simulink model "IDA_PBC"  (R2022b)
settings: Solver=FixedStepAuto  StartTime=0.0  StopTime=50  FixedStep=0.001  RelTol=1e-3
undefined symbols (not defined in the file): l_v, m_v, M_v, phi_desired, q2, q2_s
settings Model: Creator=ali14  LastModifiedBy=ali14

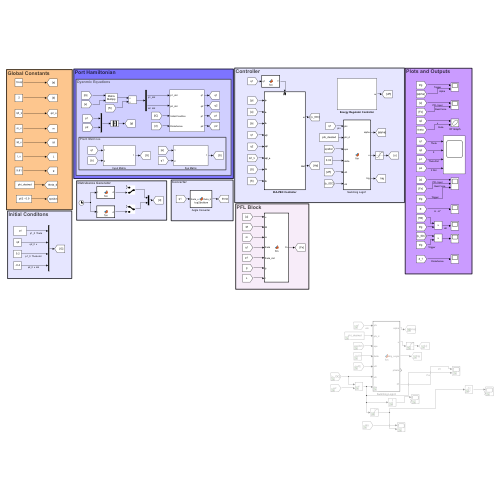
[thumbnail: Simulink's stored preview of the top-level diagram]
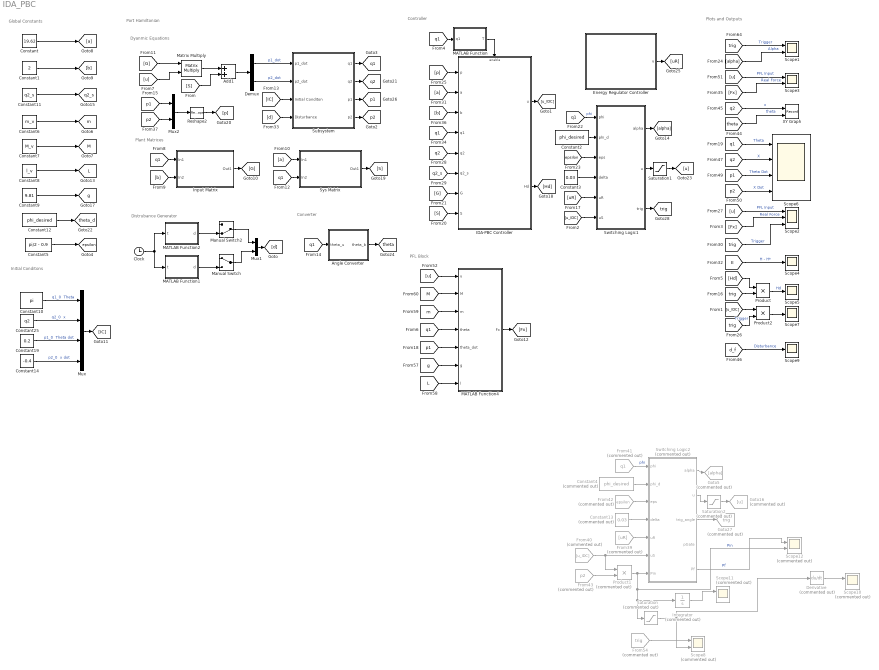
== system IDA_PBC ==
  note: Controller
  note: Plots and Outputs
  note: Initial Conditons
  note: Plant Matrices
  note: Dyanmic Equations
  note: Port Hamiltonian
  note: Converter
  note: Global Constants
  note: PFL Block
  note: Distrubance Generator
  Add1 : Sum
  Angle Converter : MATLAB Function  TreatAsAtomicUnit=on
  Clock : Clock
  Constant : Constant  Value=19.62
  Constant1 : Constant  Value=2
  Constant10 : Constant  Value=pi
  Constant11 : Constant  Value=q2_s
  Constant12 : Constant  Value=phi_desired
  Constant13 : Constant  Commented=on  Value=0.03
  Constant14 : Constant  Value=-0.4
  Constant19 : Constant  Value=0.2
  Constant2 : Constant  Value=phi_desired
  Constant25 : Constant  Value=q2
  Constant3 : Constant  Value=0.03
  Constant4 : Constant  Commented=on  Value=phi_desired
  Constant5 : Constant  Value=pi/2 - 0.9
  Constant6 : Constant  Value=m_v
  Constant7 : Constant  Value=M_v
  Constant8 : Constant  Value=l_v
  Constant9 : Constant  Value=9.81
  Demux : Demux  Outputs=2
  Derivative : Derivative  Commented=on
  Energy Regulator Controller : Subsystem
  From39 : From  Commented=on  GotoTag=uR
  From40 : From  Commented=on  GotoTag=u_IDC
  From41 : From  Commented=on  GotoTag=q1  TagVisibility=global
  From42 : From  Commented=on  GotoTag=epsilon  TagVisibility=global
  From43 : From  Commented=on  GotoTag=p2  TagVisibility=global
  From54 : From  Commented=on  GotoTag=trig  TagVisibility=global
  Goto16 : Goto  Commented=on  GotoTag=u
  Goto27 : Goto  Commented=on  GotoTag=trig  TagVisibility=global
  Goto5 : Goto  Commented=on  GotoTag=alpha
  IDA-PBC Controller : Subsystem
  Input Matrix : Subsystem
  Integrator : Integrator  Commented=on
  MATLAB Function : MATLAB Function  TreatAsAtomicUnit=on
  MATLAB Function1 : MATLAB Function  TreatAsAtomicUnit=on
  MATLAB Function2 : MATLAB Function  TreatAsAtomicUnit=on
  MATLAB Function4 : MATLAB Function  TreatAsAtomicUnit=on
  Manual Switch : ManualSwitch
  Manual Switch2 : ManualSwitch  CurrentSetting=0
  Matrix Multiply : Product  Multiplication=Matrix(*)
  Mux : Mux
  Mux1 : Mux  Inputs=2
  Mux2 : Mux  Inputs=2
  Product : Product
  Product1 : Product  Commented=on
  Product2 : Product
  Reshape2 : Reshape  OutputDimensionality=Column vector (2-D)
  Saturation : Saturate  Commented=on  UpperLimit=30  LowerLimit=-30
  Saturation1 : Saturate  UpperLimit=10  LowerLimit=-10
  Saturation2 : Saturate  Commented=on  UpperLimit=10  LowerLimit=-10
  Scope1 : Scope  NumInputPorts=2
  Scope{8,10..12} (4 alike) : Scope  Commented=on  NumInputPorts=2
  Scope2 : Scope  NumInputPorts=3
  Scope3 : Scope  NumInputPorts=2
  Scope{4..5,7,9} (4 alike) : Scope
  Scope6 : Scope  NumInputPorts=4
  Subsystem : Subsystem
  Switching Logic1 : MATLAB Function  TreatAsAtomicUnit=on
  Switching Logic2 : MATLAB Function  Commented=on  TreatAsAtomicUnit=on
  Sys Matrix : Subsystem
  XY Graph : Record  FileSettingsInternal="{\"entries\":[{\"content\":{\"excelSettings\":{\"content\":{},\"type\":\"Streamout.ExcelSettings\"}},\"type\":\"Streamout.FileSettingStorage\",\"uuid\":\"b4495491-268c-4705-8b0b-045f781b1a9d\"}],\"packageUris\":[\"http://schema.mathworks.com/mf0/streamout_blocks/R2020a\"],\"version\":\"1.0\"}"  Layout=[1 1]  SignalsInternal="{\"entries\":[{\"content\":{\"signals\":[{\"content\":{\"blockPath\":[\"IDA_PBC/XY Graph\"],\"channel\":[],\"dimensions\":[1,1],\"domain\":\"IDA_PBC/XY Graph\",\"lineColor\":\"#a2142f\",\"plots\":[1],\"port\":1,\"sid\":[\"\"],\"signalID\":19,\"signalName\":\"x\"},\"type\":\"RecordBlkView.Signal\",\"uuid\":\"3616e9f1-c643-483d-881a-894239690917\"},{\"content\":{\"blockPath\":[\"IDA_PBC/XY Graph\"],\"channel\":[],\"dimensions\":[1],\"domain\":\"IDA_PBC/XY Graph\",\"lineColor\":\"#139fff\",\"plots\":[1],\"port\":2,\"sid\":[\"\"],\"signalID\":23,\"signalName\":\"theta\"},\"type\":\"RecordBlkView.Signal\",\"uuid\":\"444c35d6-5370-4ebf-81a1-b594d5e0da69\"}]},\"type\":\"RecordBlkView.InputSignals\",\"uuid\":\"ab54f437-3e6c-482a-a295-04311a9801ac\"}],\"packageUris\":[\"http://schema.mathworks.com/mf0/streamout_blocks/R2020a\"],\"version\":\"1.0\"}"  VisualizationBindings="{\"xyplotplugin\":{\"info\":[{\"series\":[{\"bindingParametersList\":[{\"parameter\":\"X-Axis\",\"signalID\":19,\"signalName\":\"x\"},{\"parameter\":\"Y-Axis\",\"signalID\":23,\"signalName\":\"theta\"}],\"seriesID\":56537}],\"subplotID\":1}]}}"  CompatibilityTag=XY
  tag scope: L=global, M=global, epsilon=global, g=global, m=global, p1=global, p2=global, q1=global, q2=global, q2_s=global, theta=global, theta_d=global, trig=global
  wires:
  Constant/1 -> [a]
  Constant1/1 -> [b]
  [G] -> Matrix Multiply/1
  [u] -> Matrix Multiply/2
  Matrix Multiply/1 -> Add1/1
  Add1/1 -> Demux/1
  Constant11/1 -> [q2_s]
  [q2] -> XY Graph/1  "x"
  [theta] -> XY Graph/2  "theta"
  [q1] -> Scope6/1  "Theta"
  [q2] -> Scope6/2  "X"
  [p1] -> Scope6/3  "Theta Dot"
  [p2] -> Scope6/4  "X Dot"
  [u] -> Scope3/1  "PFL Input"
  [m] -> MATLAB Function4/3(m)
  [L] -> MATLAB Function4/7(l)
  [p1] -> MATLAB Function4/5(theta_dot)
  [g] -> MATLAB Function4/6(g)
  [q1] -> MATLAB Function4/4(theta)
  [M] -> MATLAB Function4/2(M)
  [u] -> MATLAB Function4/1(u)
  MATLAB Function4/1(Fx) -> [Fx]
  [G] -> IDA-PBC Controller/7(G)
  [S] -> IDA-PBC Controller/8(S)
  [p] -> IDA-PBC Controller/1(p)
  [a] -> IDA-PBC Controller/2(a)
  [b] -> IDA-PBC Controller/3(b)
  [q2_s] -> IDA-PBC Controller/6(q2_s)
  Constant7/1 -> [M]
  Constant6/1 -> [m]
  Constant8/1 -> [L]
  Constant9/1 -> [g]
  Constant12/1 -> [theta_d]
  [q1] -> Angle Converter/1(theta_u)
  Angle Converter/1(theta_b) -> [theta]
  Mux2/1 -> Reshape2/1
  Reshape2/1 -> [p]
  [p1] -> Mux2/1
  [p2] -> Mux2/2
  MATLAB Function/1(T) -> IDA-PBC Controller/Enable
  Constant5/1 -> [epsilon]
  IDA-PBC Controller/1(u) -> [u_IDC]
  [q1] -> Input Matrix/1(In1)
  [b] -> Input Matrix/2(In2)
  Input Matrix/1(Out1) -> [G]
  [a] -> Sys Matrix/1(In1)
  [q1] -> Sys Matrix/2(In2)
  Sys Matrix/1(Out1) -> [S]
  [S] -> Add1/2
  Constant25/1 -> Mux/2  "q2_0  x"
  Constant10/1 -> Mux/1  "q1_0  Theta"
  Constant19/1 -> Mux/3  "p1_0  Theta dot"
  Constant14/1 -> Mux/4  "p2_0  x dot"
  Subsystem/4(p2) -> [p2]
  Subsystem/2(q2) -> [q2]
  Subsystem/3(p1) -> [p1]
  Subsystem/1(q1) -> [q1]
  Mux/1 -> [IC]
  [IC] -> Subsystem/3(Initial Conditon)
  Demux/1 -> Subsystem/1(p1_dot)  "p1_dot"
  Demux/2 -> Subsystem/2(p2_dot)  "p2_dot"
  MATLAB Function2/1(d) -> Manual Switch2/2
  Manual Switch2/1 -> Mux1/1
  MATLAB Function1/1(d) -> Manual Switch/2
  Manual Switch/1 -> Mux1/2
  Clock/1 -> MATLAB Function2/1(t), MATLAB Function1/1(t)
  Mux1/1 -> [d]
  [d] -> Subsystem/4(Disturbance)
  [Fx] -> Scope3/2  "Real Force"
  [q1] -> IDA-PBC Controller/4(q1)
  [q2] -> IDA-PBC Controller/5(q2)
  Energy Regulator Controller/1(u) -> [uR]
  IDA-PBC Controller/2(Hd) -> [Hd]
  [q1] -> MATLAB Function/1(q1)
  Constant2/1 -> Switching Logic1/2(phi_d)
  Switching Logic1/2(u) -> Saturation1/1
  [epsilon] -> Switching Logic1/3(eps)
  Switching Logic1/1(alpha) -> [alpha]
  [q1] -> Switching Logic1/1(phi)  "phi"
  [uR] -> Switching Logic1/5(uR)
  [u_IDC] -> Switching Logic1/6(uS)
  Constant3/1 -> Switching Logic1/4(delta)
  [trig] -> Scope1/1  "Trigger"
  Switching Logic1/3(trig) -> [trig]
  [alpha] -> Scope1/2  "Alpha"
  [Fx] -> Scope2/2  "Real Force"
  [u] -> Scope2/1  "PFL Input"
  [trig] -> Scope2/3  "Trigger"
  [E] -> Scope4/1  "H - H*"
  Product/1 -> Scope5/1  "Hd"
  [trig] -> Product/2
  [Hd] -> Product/1
  Saturation1/1 -> [u]
  Switching Logic2/2(u) -> Saturation2/1
  Saturation2/1 -> Goto16/1
  From41/1 -> Switching Logic2/1(phi)  "phi"
  Constant13/1 -> Switching Logic2/4(delta)
  Switching Logic2/1(alpha) -> Goto5/1
  From39/1 -> Switching Logic2/5(uR)
  Switching Logic2/3(trig_angle) -> Goto27/1
  Constant4/1 -> Switching Logic2/2(phi_d)
  From40/1 -> Switching Logic2/6(uS), Product1/1
  From42/1 -> Switching Logic2/3(eps)
  Product1/1 -> Scope12/2, Integrator/1, Saturation/1, Switching Logic2/7(Pin)  "Pin"
  From43/1 -> Product1/2
  Saturation/1 -> Derivative/1, Scope8/2
  From54/1 -> Scope8/1
  Derivative/1 -> Scope10/1
  Integrator/1 -> Scope11/1
  Switching Logic2/5(Pf) -> Scope12/1  "Pf"
  [u_IDC] -> Product2/1
  [trig] -> Product2/2  "Trigger"
  Product2/1 -> Scope7/1
  [d_f] -> Scope9/1  "Disturbance"

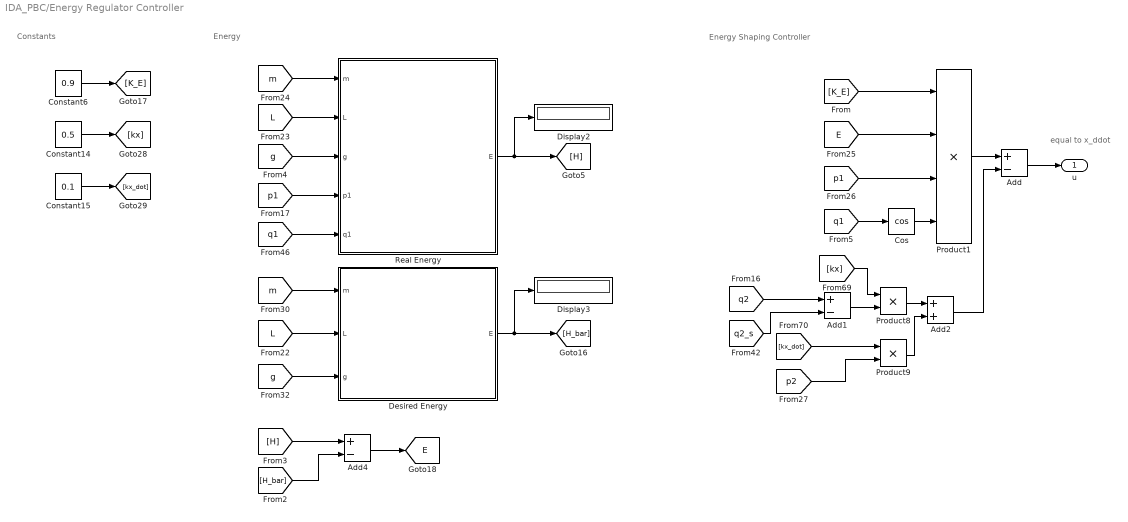
== system IDA_PBC/Energy Regulator Controller ==
  note: Energy
  note: Energy Shaping Controller
  note: Constants
  note: equal to x_ddot
  Add : Sum  Inputs=+-
  Add1 : Sum  Inputs=+-
  Add2 : Sum
  Add4 : Sum  Inputs=+-
  Constant14 : Constant  Value=0.5
  Constant15 : Constant  Value=0.1
  Constant6 : Constant  Value=0.9
  Cos : Trigonometry  Operator=cos
  Desired Energy : Subsystem
  Display2 : Display
  Display3 : Display
  Product1 : Product  Inputs=4
  Product8 : Product
  Product9 : Product
  Real Energy : Subsystem
  u : Outport
  tag scope: E=global
  wires:
  [H_bar] -> Add4/2
  [g] -> Real Energy/3(g)
  Real Energy/1(E) -> [H], Display2/1
  [m] -> Real Energy/1(m)
  [q1] -> Real Energy/5(q1)
  Desired Energy/1(E) -> [H_bar], Display3/1
  [L] -> Desired Energy/2(L)
  [m] -> Desired Energy/1(m)
  [L] -> Real Energy/2(L)
  [H] -> Add4/1
  Add4/1 -> [E]
  [p1] -> Real Energy/4(p1)
  [g] -> Desired Energy/3(g)
  Add/1 -> u/1
  [q2_s] -> Add1/2
  [q2] -> Add1/1
  Add1/1 -> Product8/2
  Constant15/1 -> [kx_dot]
  Constant14/1 -> [kx]
  Add2/1 -> Add/2
  [K_E] -> Product1/1
  [E] -> Product1/2
  [p1] -> Product1/3
  [kx_dot] -> Product9/1
  Product1/1 -> Add/1
  Constant6/1 -> [K_E]
  Cos/1 -> Product1/4
  [p2] -> Product9/2
  [kx] -> Product8/1
  Product9/1 -> Add2/2
  Product8/1 -> Add2/1
  [q1] -> Cos/1

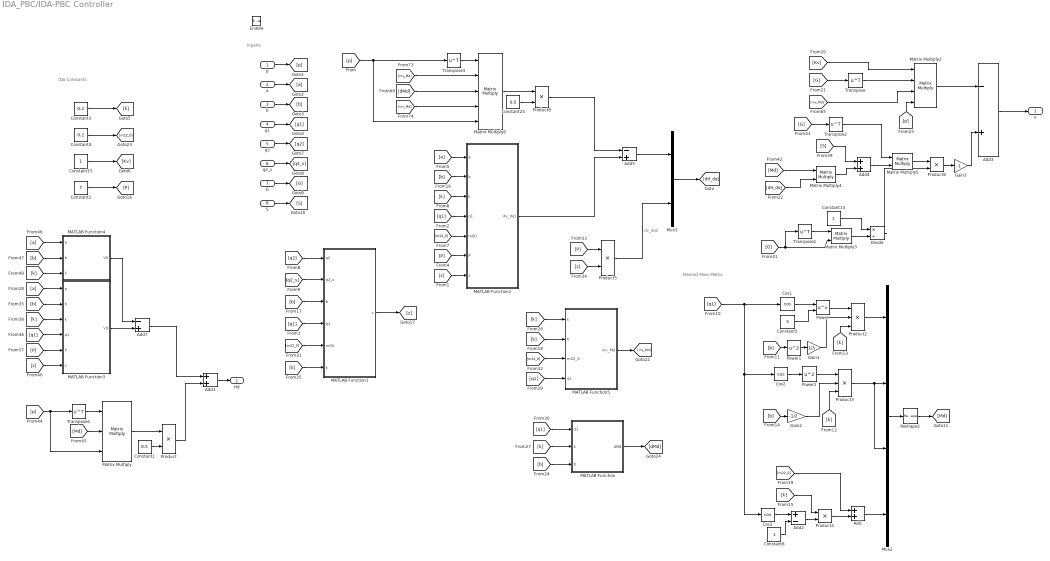
== system IDA_PBC/IDA-PBC Controller ==
  note: Inports
  note: Desired Mass Matrix
  note: IDA Constants
  p : Inport
  a : Inport  Port=2
  b : Inport  Port=3
  q1 : Inport  Port=4
  q2 : Inport  Port=5
  q2_s : Inport  Port=6
  G : Inport  Port=7
  S : Inport  Port=8
  Enable : EnablePort
  Add : Sum
  Add1 : Sum
  Add2 : Sum  Inputs=+-
  Add3 : Sum  Inputs=-+
  Add4 : Sum
  Add5 : Sum  Inputs=-+
  Add7 : Sum  Inputs=-+
  Constant1 : Constant  Value=0.5
  Constant13 : Constant
  Constant15 : Constant
  Constant2 : Constant  Value=7
  Constant24 : Constant  Value=0.5
  Constant3 : Constant  Value=0.2
  Constant4 : Constant  Value=0.2
  Constant5 : Constant  Value=3
  Constant8 : Constant
  Cos1 : Trigonometry  Operator=cos
  Cos2 : Trigonometry  Operator=cos
  Cos3 : Trigonometry  Operator=cos
  Divide : Product  Inputs=*/
  Gain1 : Gain  Gain=1/3
  Gain2 : Gain  Gain=-1/2
  Gain3 : Gain  Gain=-1
  MATLAB Function : MATLAB Function  TreatAsAtomicUnit=on
  MATLAB Function1 : MATLAB Function  TreatAsAtomicUnit=on
  MATLAB Function2 : MATLAB Function  TreatAsAtomicUnit=on
  MATLAB Function3 : MATLAB Function  TreatAsAtomicUnit=on
  MATLAB Function4 : MATLAB Function  TreatAsAtomicUnit=on
  MATLAB Function5 : MATLAB Function  TreatAsAtomicUnit=on
  Matrix Multiply : Product  Inputs=3  Multiplication=Matrix(*)
  Matrix Multiply2 : Product  Inputs=4  Multiplication=Matrix(*)
  Matrix Multiply3 : Product  Multiplication=Matrix(*)
  Matrix Multiply4 : Product  Multiplication=Matrix(*)
  Matrix Multiply5 : Product  Multiplication=Matrix(*)
  Matrix Multiply6 : Product  Inputs=5  Multiplication=Matrix(*)
  Mux2 : Mux
  Mux3 : Mux  Inputs=2
  Power : Math  Operator=pow
  Power1 : Math  Operator=square
  Power2 : Math  Operator=square
  Product{,4..6,8} (5 alike) : Product
  Product2 : Product  Inputs=3
  Product3 : Product  Inputs=3
  Reshape2 : Reshape  OutputDimensionality=Customize  OutputDimensions=[2,2]
  Transpose{,1..4} (5 alike) : Math  Operator=transpose
  u : Outport
  Hd : Outport  Port=2
  wires:
  Product5/1 -> Mux3/2  "dv_dq2"
  MATLAB Function1/1(z) -> [z]
  Add5/1 -> Mux3/1
  [a] -> MATLAB Function2/1(a)
  MATLAB Function/1(dMd) -> [dMd]
  MATLAB Function5/1(inv_Md) -> [inv_Md]
  [q2] -> MATLAB Function1/1(q2)
  [q2_s] -> MATLAB Function1/2(q2_s)
  Mux3/1 -> [dH_dq]
  [z] -> MATLAB Function2/7(z)
  Matrix Multiply6/1 -> Product8/1
  [dMd] -> Matrix Multiply6/3
  [inv_Md] -> Matrix Multiply6/2
  [inv_Md] -> Matrix Multiply6/4
  Transpose3/1 -> Matrix Multiply6/1
  [p] -> Transpose3/1, Matrix Multiply6/5
  Constant24/1 -> Product8/2
  Product8/1 -> Add5/1
  MATLAB Function2/1(dv_dq1) -> Add5/2
  Divide/1 -> Product6/2
  [inv_Md] -> Matrix Multiply2/3
  [G] -> Transpose/1
  [S] -> Add4/1
  Transpose1/1 -> Matrix Multiply3/1
  [p] -> Matrix Multiply2/4
  Product6/1 -> Gain3/1
  Add3/1 -> u/1
  Transpose/1 -> Matrix Multiply2/2
  Matrix Multiply3/1 -> Divide/2
  [dH_dq] -> Matrix Multiply4/2
  Add4/1 -> Matrix Multiply5/2
  Transpose2/1 -> Matrix Multiply5/1
  [Md] -> Matrix Multiply4/1
  Matrix Multiply4/1 -> Add4/2
  Constant13/1 -> Divide/1
  Gain3/1 -> Add3/2
  [Kv] -> Matrix Multiply2/1
  Matrix Multiply5/1 -> Product6/1
  [G] -> Transpose1/1, Matrix Multiply3/2
  [G] -> Transpose2/1
  Matrix Multiply2/1 -> Add3/1
  p/1 -> [p]
  a/1 -> [a]
  b/1 -> [b]
  q2_s/1 -> [q2_s]
  G/1 -> [G]
  S/1 -> [S]
  Power/1 -> Product2/1
  Product2/1 -> Mux2/1
  Power2/1 -> Product3/1
  Cos1/1 -> Power/1
  Power1/1 -> Gain1/1
  Cos3/1 -> Add2/1
  [b] -> Power1/1
  [q1] -> Cos3/1, Cos2/1, Cos1/1
  Product4/1 -> Add/2
  Reshape2/1 -> [Md]
  Constant5/1 -> Power/2
  [k] -> Product4/1
  Constant8/1 -> Add2/2
  Gain2/1 -> Product3/2
  [k] -> Product2/3
  Cos2/1 -> Power2/1
  Product3/1 -> Mux2/3, Mux2/2
  [b] -> Gain2/1
  Add2/1 -> Product4/2
  Gain1/1 -> Product2/2
  Mux2/1 -> Reshape2/1
  [m22_0] -> Add/1
  Add/1 -> Mux2/4
  [k] -> Product3/3
  [b] -> MATLAB Function2/2(b)
  [b] -> MATLAB Function1/3(b)
  [b] -> MATLAB Function5/2(b)
  [b] -> MATLAB Function/3(b)
  [k] -> MATLAB Function2/3(k)
  [k] -> MATLAB Function1/6(k)
  [k] -> MATLAB Function5/1(k)
  [k] -> MATLAB Function/2(k)
  [q1] -> MATLAB Function2/4(q1)
  [q1] -> MATLAB Function1/4(q1)
  [q1] -> MATLAB Function5/4(q1)
  [q1] -> MATLAB Function/1(q1)
  [m22_0] -> MATLAB Function2/5(m00)
  [m22_0] -> MATLAB Function1/5(m00)
  [m22_0] -> MATLAB Function5/3(m22_0)
  [P] -> Product5/1
  [P] -> MATLAB Function2/6(P)
  [z] -> Product5/2
  q1/1 -> [q1]
  q2/1 -> [q2]
  Constant3/1 -> [k]
  Constant15/1 -> [Kv]
  Constant4/1 -> [m22_0]
  Constant2/1 -> [P]
  [k] -> MATLAB Function3/3(k)
  [a] -> MATLAB Function3/1(a)
  [b] -> MATLAB Function3/2(b)
  [q1] -> MATLAB Function3/4(q1)
  [P] -> MATLAB Function3/5(P)
  [z] -> MATLAB Function3/6(z)
  Matrix Multiply/1 -> Product/1
  Constant1/1 -> Product/2
  Transpose4/1 -> Matrix Multiply/1
  [p] -> Transpose4/1, Matrix Multiply/3
  [Md] -> Matrix Multiply/2
  Product/1 -> Add1/2
  Add1/1 -> Hd/1
  [a] -> MATLAB Function4/1(a)
  [b] -> MATLAB Function4/2(b)
  [k] -> MATLAB Function4/3(k)
  MATLAB Function3/1(Vd) -> Add7/2
  Add7/1 -> Add1/1
  MATLAB Function4/1(V0) -> Add7/1

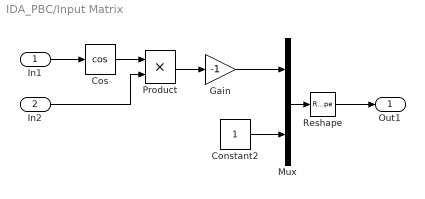
== system IDA_PBC/Input Matrix ==
  In1 : Inport
  In2 : Inport  Port=2
  Constant2 : Constant
  Cos : Trigonometry  Operator=cos
  Gain : Gain  Gain=-1
  Mux : Mux  Inputs=2
  Product : Product
  Reshape : Reshape  OutputDimensionality=Column vector (2-D)
  Out1 : Outport
  wires:
  Cos/1 -> Product/1
  Mux/1 -> Reshape/1
  Product/1 -> Gain/1
  Constant2/1 -> Mux/2
  In1/1 -> Cos/1
  Gain/1 -> Mux/1
  In2/1 -> Product/2
  Reshape/1 -> Out1/1

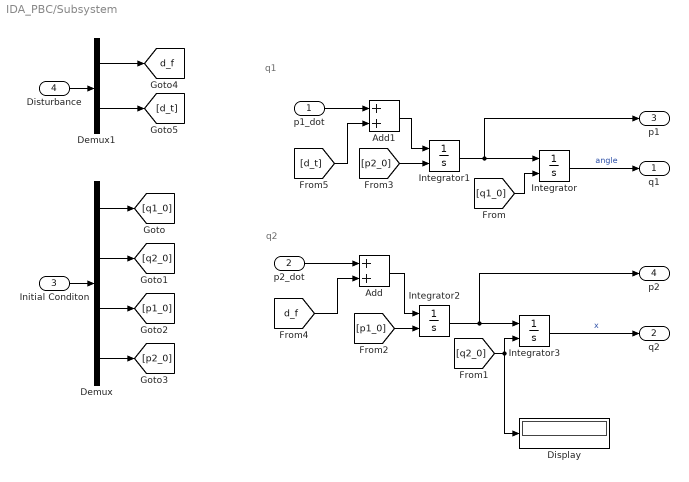
== system IDA_PBC/Subsystem ==
  note: q2
  note: q1
  p1_dot : Inport
  p2_dot : Inport  Port=2
  Initial Conditon : Inport  Port=3
  Disturbance : Inport  Port=4
  Add : Sum
  Add1 : Sum
  Demux : Demux
  Demux1 : Demux  Outputs=2
  Display : Display
  Integrator : Integrator  InitialConditionSource=external  WrapState=on
  Integrator1 : Integrator  InitialConditionSource=external
  Integrator2 : Integrator  InitialConditionSource=external
  Integrator3 : Integrator  InitialConditionSource=external
  q1 : Outport
  q2 : Outport  Port=2
  p1 : Outport  Port=3
  p2 : Outport  Port=4
  tag scope: d_f=global
  wires:
  Add/1 -> Integrator2/1
  Integrator3/1 -> q2/1  "x"
  Integrator2/1 -> p2/1, Integrator3/1
  Integrator1/1 -> p1/1, Integrator/1
  Integrator/1 -> q1/1  "angle"
  Initial Conditon/1 -> Demux/1
  Disturbance/1 -> Demux1/1
  Demux/1 -> [q1_0]
  [q1_0] -> Integrator/2
  Demux/2 -> [q2_0]
  Demux/3 -> [p1_0]
  Demux/4 -> [p2_0]
  [q2_0] -> Display/1, Integrator3/2
  Add1/1 -> Integrator1/1
  p1_dot/1 -> Add1/1
  p2_dot/1 -> Add/1
  Demux1/2 -> [d_t]
  [d_f] -> Add/2
  [d_t] -> Add1/2
  [p1_0] -> Integrator2/2
  [p2_0] -> Integrator1/2
  Demux1/1 -> [d_f]

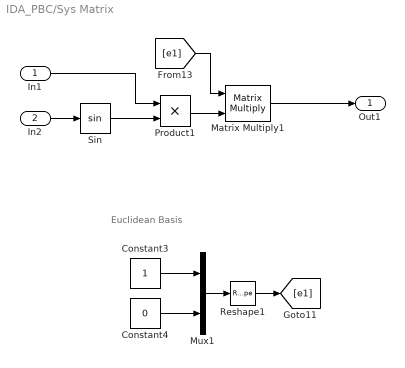
== system IDA_PBC/Sys Matrix ==
  note: Euclidean Basis
  In1 : Inport
  In2 : Inport  Port=2
  Constant3 : Constant
  Constant4 : Constant  Value=0
  Matrix Multiply1 : Product  Multiplication=Matrix(*)
  Mux1 : Mux  Inputs=2
  Product1 : Product
  Reshape1 : Reshape  OutputDimensionality=Column vector (2-D)
  Sin : Trigonometry
  Out1 : Outport
  wires:
  [e1] -> Matrix Multiply1/1
  Product1/1 -> Matrix Multiply1/2
  Sin/1 -> Product1/2
  In1/1 -> Product1/1
  In2/1 -> Sin/1
  Matrix Multiply1/1 -> Out1/1
  Constant4/1 -> Mux1/2
  Constant3/1 -> Mux1/1
  Reshape1/1 -> [e1]
  Mux1/1 -> Reshape1/1

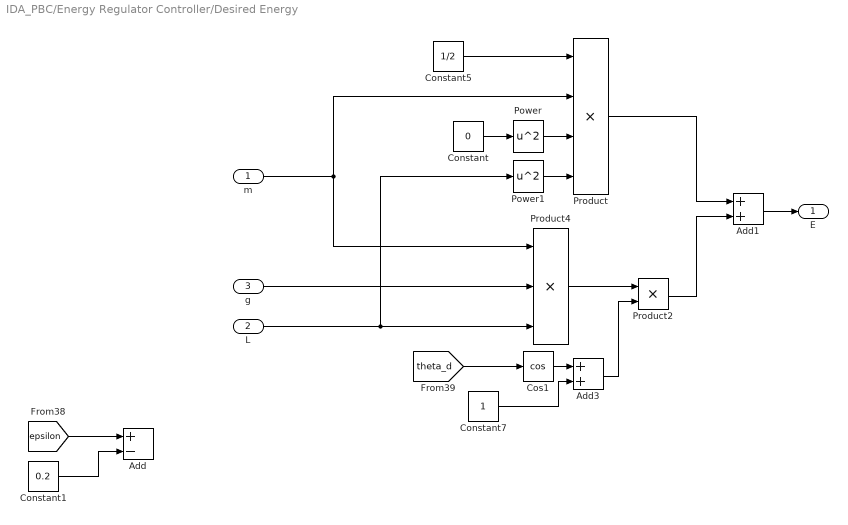
== system IDA_PBC/Energy Regulator Controller/Desired Energy ==
  m : Inport
  L : Inport  Port=2
  g : Inport  Port=3
  Add : Sum  Inputs=+-
  Add1 : Sum
  Add3 : Sum
  Constant : Constant  Value=0
  Constant1 : Constant  Value=0.2
  Constant5 : Constant  Value=1/2
  Constant7 : Constant
  Cos1 : Trigonometry  Operator=cos
  Power : Math  Operator=square
  Power1 : Math  Operator=square
  Product : Product  Inputs=4
  Product2 : Product
  Product4 : Product  Inputs=3
  E : Outport
  wires:
  Product4/1 -> Product2/1
  Power/1 -> Product/3
  Constant7/1 -> Add3/2
  m/1 -> Product4/1, Product/2
  Constant/1 -> Power/1
  Product/1 -> Add1/1
  Cos1/1 -> Add3/1
  Add3/1 -> Product2/2
  Power1/1 -> Product/4
  Product2/1 -> Add1/2
  Constant5/1 -> Product/1
  Add1/1 -> E/1
  g/1 -> Product4/2
  L/1 -> Power1/1, Product4/3
  [theta_d] -> Cos1/1
  Constant1/1 -> Add/2
  [epsilon] -> Add/1

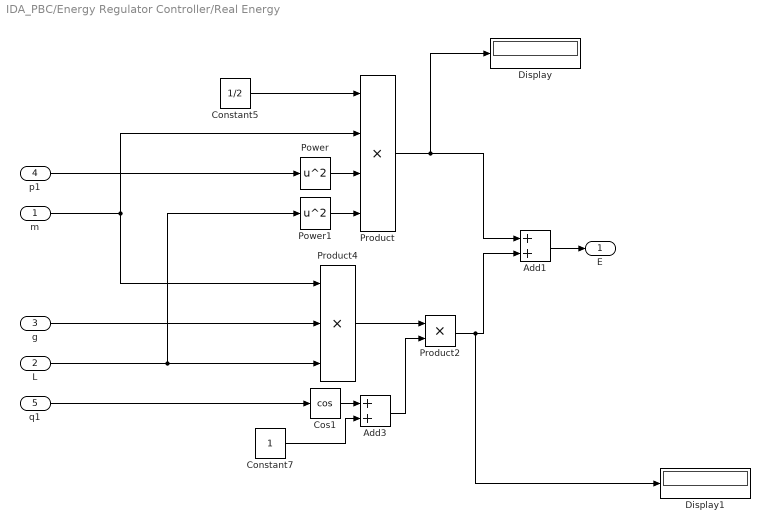
== system IDA_PBC/Energy Regulator Controller/Real Energy ==
  m : Inport
  L : Inport  Port=2
  g : Inport  Port=3
  p1 : Inport  Port=4
  q1 : Inport  Port=5
  Add1 : Sum
  Add3 : Sum
  Constant5 : Constant  Value=1/2
  Constant7 : Constant
  Cos1 : Trigonometry  Operator=cos
  Display : Display
  Display1 : Display
  Power : Math  Operator=square
  Power1 : Math  Operator=square
  Product : Product  Inputs=4
  Product2 : Product
  Product4 : Product  Inputs=3
  E : Outport
  wires:
  Product4/1 -> Product2/1
  Power/1 -> Product/3
  Constant7/1 -> Add3/2
  m/1 -> Product4/1, Product/2
  p1/1 -> Power/1
  Product/1 -> Display/1, Add1/1
  Cos1/1 -> Add3/1
  Add3/1 -> Product2/2
  Power1/1 -> Product/4
  Product2/1 -> Display1/1, Add1/2
  q1/1 -> Cos1/1
  Constant5/1 -> Product/1
  Add1/1 -> E/1
  g/1 -> Product4/2
  L/1 -> Power1/1, Product4/3

== matlab function IDA_PBC/MATLAB Function1 ==
  data: t input; d output
function d = fcn(t)
if and(t > 20 , t <30)
    d = 2 + 4*sin(10*t);
else
    d = 0;
end

== matlab function IDA_PBC/MATLAB Function2 ==
  data: t input; d output
function d = fcn(t)
if and(t > 10 , t <10.5)
    d = 3;
elseif and(t>15 , t <16)
    d = 5;
elseif and(t>20 , t <20.5)
    d = -12;
else
    d = 0;
end

== matlab function IDA_PBC/MATLAB Function ==
  data: q1 input; T output
function T = fcn(q1)

if and(q1 > -pi/2 + 0.1 , q1 < pi/2 - 0.1) 
    T = 1;
else
    T = 0;
end

== matlab function IDA_PBC/MATLAB Function4 ==
  data: u input; Fx output; M input; m input; theta input; theta_dot input; g input; l input
function Fx = fcn(u , M ,m ,theta,theta_dot,g,l)

Fx = u*(M+m*sin(theta)^2) + ...
(m*l*sin(theta)*theta_dot^2 - m*g*sin(theta)*cos(theta));

== matlab function IDA_PBC/IDA-PBC Controller/MATLAB Function4 ==
  data: a input; V0 output; b input; k input
function V0 = fcn(a , b,k)
V0 = (3*a)/(k*b^2);

== matlab function IDA_PBC/Switching Logic1 ==
  settings: updateMethod=DISCRETE
  data: phi input; phi_d input; eps input; delta input; alpha output; u output; uR input; uS input; trig output
function [alpha,u,trig] = fcn(phi, phi_d, eps, delta, uR, uS)
% Smooth switching (blending) between uR and uS
% eps   : half-width of switching region (your eps = pi/2 - 0.7)
% delta : smoothing width inside eps (choose e.g. 0.05~0.15 rad)

d = abs(phi - phi_d);

% Clamp delta to safe range (avoid divide-by-zero)
delta = max(delta, 1e-6);

% Define a smooth transition band: [eps-delta, eps+delta]
d1 = eps - delta;
d2 = eps + delta;

if d <= d1
    alpha = 1;      % fully stabilizer uS
    trig  = 1;
elseif d >= d2
    alpha = 0;      % fully regulator uR
    trig  = 0;
else
    % Smoothstep from 1 -> 0 over [d1, d2]
    t = (d - d1) / (d2 - d1);   % t in (0,1)
    s = t^2*(3 - 2*t);          % smoothstep (C1)
    alpha = 1 - s;
    trig  = 1;
end

u = (1 - alpha)*uR + alpha*uS;
end

== matlab function IDA_PBC/IDA-PBC Controller/MATLAB Function1 ==
  data: q2 input; z output; q2_s input; b input; q1 input; m00 input; k input
function z = fcn(q2,q2_s,b,q1,m00,k)
z = (q2 - q2_s) ...
    + (3/b)*log(1./cos(q1) + tan(q1))*2.302585 ...
    + (6*m00/(k*b))*tan(q1);
end

== matlab function IDA_PBC/IDA-PBC Controller/MATLAB Function ==
  data: q1 input; dMd output; k input; b input
function dMd = dMd_dq1(q1, k, b)
% dMd_dq1  Computes ∂Md/∂q1 for the IDA-PBC pendulum-cart system
%
% Inputs:
%   q1  - pendulum angle (rad)
%   k   - design parameter k
%   b   - system parameter b
%
% Output:
%   dMd - 2x2 matrix ∂Md/∂q1

c = cos(q1);
s = sin(q1);

dMd = [ -k*b^2*c^2*s,     k*b*c*s;
         k*b*c*s,        -k*s       ];
end

== matlab function IDA_PBC/IDA-PBC Controller/MATLAB Function2 ==
  data: a input; dv_dq1 output; b input; k input; q1 input; m00 input; P input; z input
function dv_dq1 = fcn(a,b,k,q1,m00,P,z)

term1 = (6*a*sin(q1)) / (k*b^2*cos(q1)^3);
term2 = P*z * ( 3/(b*cos(q1)) + 6*m00/(k*b*cos(q1)^2) );

dv_dq1 = term1 + term2;

end

== matlab function IDA_PBC/IDA-PBC Controller/MATLAB Function5 ==
  data: k input; inv_Md output; b input; m22_0 input; q1 input
function inv_Md = fcn(k,b,m22_0,q1)

det_Md = (k*b^2*cos(q1)^3)/3 * (m22_0 + k*(0.25*cos(q1) - 1));

adj_Md = [k*(cos(q1)-1)+m22_0  k*b*cos(q1)^2/2;
          k*b*cos(q1)^2/2      k*b^2*cos(q1)^3/3];
inv_Md = adj_Md/det_Md;

== matlab function IDA_PBC/Angle Converter ==
  data: theta_u input; theta_b output
function theta_b = top2bottom(theta_u)
%TOP2BOTTOM Convert pendulum angle from top-reference to bottom-reference
%
%   theta_u : angle measured from upright (rad), CCW positive
%   theta_b : angle measured from downward (rad), CCW positive
%
%   Output is wrapped to (-pi, pi]

    theta_b = wrapToPi(theta_u + pi);

end

== matlab function IDA_PBC/Switching Logic2 ==
  settings: updateMethod=DISCRETE
  data: phi input; phi_d input; eps input; delta input; alpha output; u output; uR input; uS input; trig_angle output; Pin input; pGate output; Pf output
function [alpha,u,trig_angle,pGate,Pf] = fcn(phi, phi_d, eps, delta, uR, uS, Pin)

Ts = 0.0001;

Pin_on_low  = -0.5;
Pin_on_high =  0.5;

Pin_off_low  = -40;
Pin_off_high =  40;

dwell_time = 0.01;
N_dwell = round(dwell_time / Ts);

tau = 0.2;
a = exp(-Ts/tau);

persistent powerGate Pf_state cnt_inband
if isempty(powerGate)
    powerGate=false; Pf_state=0; cnt_inband=0;
end

% --- Filter always computed, but used only for OFF decision (when enabled)
Pf_state = a*Pf_state + (1-a)*Pin;
Pf = Pf_state;

% --- Angle logic
d = abs(phi - phi_d);
delta = max(delta, 1e-6);
d1 = eps - delta; d2 = eps + delta;

if d <= d1
    alpha=1; trig_angle=1;
elseif d >= d2
    alpha=0; trig_angle=0;
else
    t=(d-d1)/(d2-d1); s=t^2*(3-2*t);
    alpha=1-s; trig_angle=1;
end

% --- Power gate only if in angle switching region
if trig_angle==1

    if powerGate
        % OFF decision uses FILTERED Pf (robust to spikes)
        if (Pf < Pin_off_low) || (Pf > Pin_off_high)
            powerGate = false;
            cnt_inband = 0;
        end
    else
        % ON decision uses RAW Pin (fast + strict)
        if (Pin >= Pin_on_low) && (Pin <= Pin_on_high)
            cnt_inband = cnt_inband + 1;
            if cnt_inband >= N_dwell
                powerGate = true;
                cnt_inband = 0;
            end
        else
            cnt_inband = 0;
        end
    end

    if ~powerGate
        alpha = 0;
    end

else
    cnt_inband = 0;
end

pGate = powerGate;
u = (1-alpha)*uR + alpha*uS;

end

== matlab function IDA_PBC/IDA-PBC Controller/MATLAB Function3 ==
  data: a input; Vd output; b input; k input; q1 input; P input; z input
function Vd = fcn(a ,b, k ,q1 ,P ,z)
Vd = (3*a) ./ (k .* b^2 .* cos(q1).^2) ...
     + (P/2) .* (z.^2);
